simulink model "Behavioral_Buck_Converter"  (R2026a)
settings: Solver=VariableStepAuto  StopTime=2

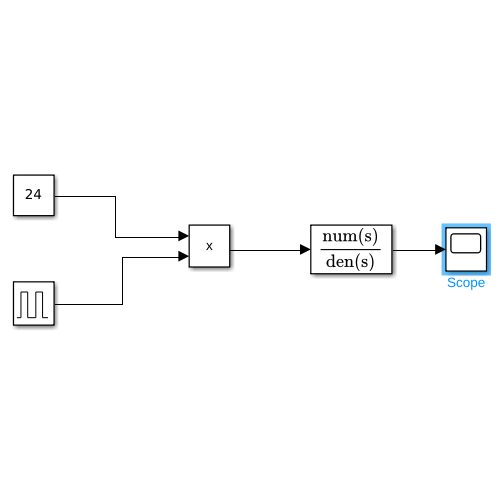
[thumbnail: Simulink's stored preview of the top-level diagram]
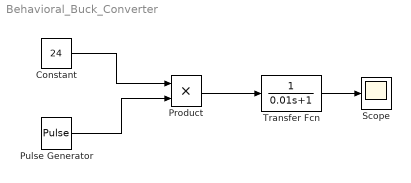
== system Behavioral_Buck_Converter ==
  Constant : Constant  Value=24
  Product : Product
  Pulse Generator : DiscretePulseGenerator  PulseType=Time based  PulseWidth=50
  Scope : Scope
      settings: ActiveDisplayYMinimum=-94.9609622186933  ActiveDisplayYMaximum=137.15286096631252
  Transfer Fcn : TransferFcn  Denominator=[0.01 1]
  wires:
  Constant/1 -> Product/1
  Pulse Generator/1 -> Product/2
  Product/1 -> Transfer Fcn/1
  Transfer Fcn/1 -> Scope/1
